simulink model "CAN1_Net_Sim"  (R2026b)
settings: Solver=VariableStepAuto
undefined symbols (not defined in the file or in its folder): P, Ts
libraries: simulink x36
settings Model: Creator=aomar  LastModifiedBy=aomar

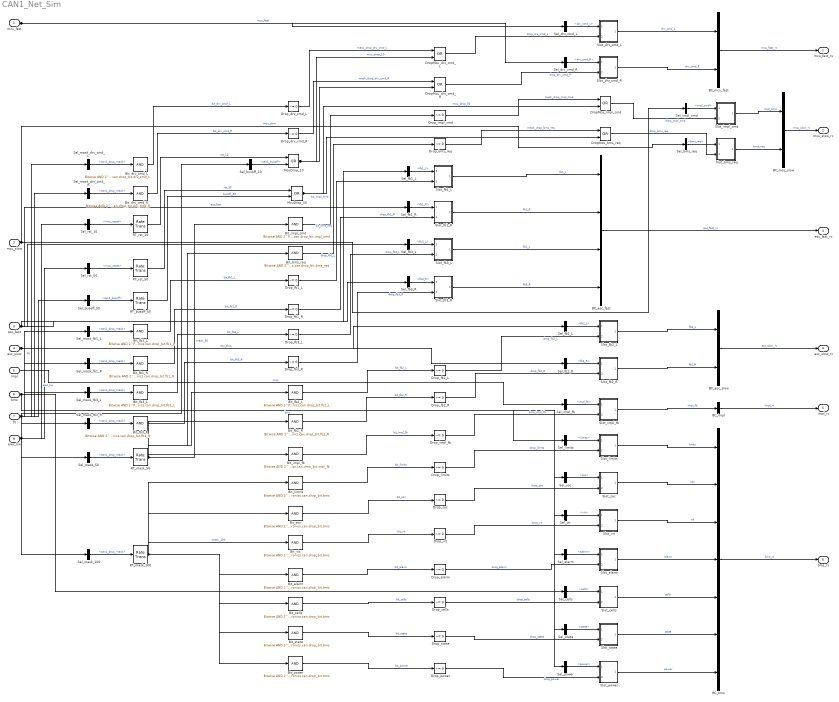
== system CAN1_Net_Sim ==
  mcu_fast : Inport  OutDataTypeStr=Bus: Bus_Can1_McuFast  SampleTime=Ts.ctrl
  mcu_slow : Inport  Port=2  OutDataTypeStr=Bus: Bus_Can1_McuSlow  SampleTime=Ts.comm
  esc_fast : Inport  Port=3  OutDataTypeStr=Bus: Bus_Can1_EscFast  SampleTime=Ts.ctrl
  esc_slow : Inport  Port=4  OutDataTypeStr=Bus: Bus_Can1_EscSlow  SampleTime=Ts.comm
  impl : Inport  Port=5  OutDataTypeStr=Bus: Bus_Can1_Impl  SampleTime=Ts.comm
  bms : Inport  Port=6  OutDataTypeStr=Bus: Bus_Can1_Bms  SampleTime=Ts.hk
  flt : Inport  Port=7  OutDataTypeStr=Bus: Bus_FaultInject  SampleTime=Ts.ctrl
  elec_hw : Inport  Port=8  OutDataTypeStr=Bus: Bus_ElecHwIn  SampleTime=Ts.base
  BC_bms : BusCreator  Inputs=7  OutDataTypeStr=Bus: Bus_Can1_Bms  NonVirtualBus=on
      settings: InheritFromInputs=off
  BC_esc_fast : BusCreator  Inputs=4  OutDataTypeStr=Bus: Bus_Can1_EscFast  NonVirtualBus=on
      settings: InheritFromInputs=off
  BC_esc_slow : BusCreator  Inputs=2  OutDataTypeStr=Bus: Bus_Can1_EscSlow  NonVirtualBus=on
      settings: InheritFromInputs=off
  BC_impl : BusCreator  Inputs=1  OutDataTypeStr=Bus: Bus_Can1_Impl  NonVirtualBus=on
      settings: InheritFromInputs=off
  BC_mcu_fast : BusCreator  Inputs=2  OutDataTypeStr=Bus: Bus_Can1_McuFast  NonVirtualBus=on
      settings: InheritFromInputs=off
  BC_mcu_slow : BusCreator  Inputs=2  OutDataTypeStr=Bus: Bus_Can1_McuSlow  NonVirtualBus=on
      settings: InheritFromInputs=off
  Bit_alarm : simulink/Logic and Bit Operations/Bitwise Operator  logicop=AND  UseBitMask=on  BitMask=2^P.electronics.can.drop_bit.bms  BitMaskRealWorld=Stored Integer
  Bit_bms_req : simulink/Logic and Bit Operations/Bitwise Operator  logicop=AND  UseBitMask=on  BitMask=2^P.electronics.can.drop_bit.bms_req  BitMaskRealWorld=Stored Integer
  Bit_cells : simulink/Logic and Bit Operations/Bitwise Operator  logicop=AND  UseBitMask=on  BitMask=2^P.electronics.can.drop_bit.bms  BitMaskRealWorld=Stored Integer
  Bit_drv_cmd_L : simulink/Logic and Bit Operations/Bitwise Operator  logicop=AND  UseBitMask=on  BitMask=2^P.electronics.can.drop_bit.drv_cmd_L  BitMaskRealWorld=Stored Integer
  Bit_drv_cmd_R : simulink/Logic and Bit Operations/Bitwise Operator  logicop=AND  UseBitMask=on  BitMask=2^P.electronics.can.drop_bit.drv_cmd_R  BitMaskRealWorld=Stored Integer
  Bit_fb1_L : simulink/Logic and Bit Operations/Bitwise Operator  logicop=AND  UseBitMask=on  BitMask=2^P.electronics.can.drop_bit.fb1_L  BitMaskRealWorld=Stored Integer
  Bit_fb1_R : simulink/Logic and Bit Operations/Bitwise Operator  logicop=AND  UseBitMask=on  BitMask=2^P.electronics.can.drop_bit.fb1_R  BitMaskRealWorld=Stored Integer
  Bit_fb2_L : simulink/Logic and Bit Operations/Bitwise Operator  logicop=AND  UseBitMask=on  BitMask=2^P.electronics.can.drop_bit.fb2_L  BitMaskRealWorld=Stored Integer
  Bit_fb2_R : simulink/Logic and Bit Operations/Bitwise Operator  logicop=AND  UseBitMask=on  BitMask=2^P.electronics.can.drop_bit.fb2_R  BitMaskRealWorld=Stored Integer
  Bit_fb3_L : simulink/Logic and Bit Operations/Bitwise Operator  logicop=AND  UseBitMask=on  BitMask=2^P.electronics.can.drop_bit.fb3_L  BitMaskRealWorld=Stored Integer
  Bit_fb3_R : simulink/Logic and Bit Operations/Bitwise Operator  logicop=AND  UseBitMask=on  BitMask=2^P.electronics.can.drop_bit.fb3_R  BitMaskRealWorld=Stored Integer
  Bit_impl_cmd : simulink/Logic and Bit Operations/Bitwise Operator  logicop=AND  UseBitMask=on  BitMask=2^P.electronics.can.drop_bit.impl_cmd  BitMaskRealWorld=Stored Integer
  Bit_impl_fb : simulink/Logic and Bit Operations/Bitwise Operator  logicop=AND  UseBitMask=on  BitMask=2^P.electronics.can.drop_bit.impl_fb  BitMaskRealWorld=Stored Integer
  Bit_limits : simulink/Logic and Bit Operations/Bitwise Operator  logicop=AND  UseBitMask=on  BitMask=2^P.electronics.can.drop_bit.bms  BitMaskRealWorld=Stored Integer
  Bit_power : simulink/Logic and Bit Operations/Bitwise Operator  logicop=AND  UseBitMask=on  BitMask=2^P.electronics.can.drop_bit.bms  BitMaskRealWorld=Stored Integer
  Bit_soc : simulink/Logic and Bit Operations/Bitwise Operator  logicop=AND  UseBitMask=on  BitMask=2^P.electronics.can.drop_bit.bms  BitMaskRealWorld=Stored Integer
  Bit_state : simulink/Logic and Bit Operations/Bitwise Operator  logicop=AND  UseBitMask=on  BitMask=2^P.electronics.can.drop_bit.bms  BitMaskRealWorld=Stored Integer
  Bit_vit : simulink/Logic and Bit Operations/Bitwise Operator  logicop=AND  UseBitMask=on  BitMask=2^P.electronics.can.drop_bit.bms  BitMaskRealWorld=Stored Integer
  DropMcu_bms_req : Logic  Operator=OR  AllPortsSameDT=off  OutDataTypeStr=boolean
  DropMcu_drv_cmd_L : Logic  Operator=OR  AllPortsSameDT=off  OutDataTypeStr=boolean
  DropMcu_drv_cmd_R : Logic  Operator=OR  AllPortsSameDT=off  OutDataTypeStr=boolean
  DropMcu_impl_cmd : Logic  Operator=OR  AllPortsSameDT=off  OutDataTypeStr=boolean
  Drop_alarm : simulink/Logic and Bit Operations/Compare To Zero  relop=~=  OutDataTypeStr=boolean
  Drop_bms_req : simulink/Logic and Bit Operations/Compare To Zero  relop=~=  OutDataTypeStr=boolean
  Drop_cells : simulink/Logic and Bit Operations/Compare To Zero  relop=~=  OutDataTypeStr=boolean
  Drop_drv_cmd_L : simulink/Logic and Bit Operations/Compare To Zero  relop=~=  OutDataTypeStr=boolean
  Drop_drv_cmd_R : simulink/Logic and Bit Operations/Compare To Zero  relop=~=  OutDataTypeStr=boolean
  Drop_fb1_L : simulink/Logic and Bit Operations/Compare To Zero  relop=~=  OutDataTypeStr=boolean
  Drop_fb1_R : simulink/Logic and Bit Operations/Compare To Zero  relop=~=  OutDataTypeStr=boolean
  Drop_fb2_L : simulink/Logic and Bit Operations/Compare To Zero  relop=~=  OutDataTypeStr=boolean
  Drop_fb2_R : simulink/Logic and Bit Operations/Compare To Zero  relop=~=  OutDataTypeStr=boolean
  Drop_fb3_L : simulink/Logic and Bit Operations/Compare To Zero  relop=~=  OutDataTypeStr=boolean
  Drop_fb3_R : simulink/Logic and Bit Operations/Compare To Zero  relop=~=  OutDataTypeStr=boolean
  Drop_impl_cmd : simulink/Logic and Bit Operations/Compare To Zero  relop=~=  OutDataTypeStr=boolean
  Drop_impl_fb : simulink/Logic and Bit Operations/Compare To Zero  relop=~=  OutDataTypeStr=boolean
  Drop_limits : simulink/Logic and Bit Operations/Compare To Zero  relop=~=  OutDataTypeStr=boolean
  Drop_power : simulink/Logic and Bit Operations/Compare To Zero  relop=~=  OutDataTypeStr=boolean
  Drop_soc : simulink/Logic and Bit Operations/Compare To Zero  relop=~=  OutDataTypeStr=boolean
  Drop_state : simulink/Logic and Bit Operations/Compare To Zero  relop=~=  OutDataTypeStr=boolean
  Drop_vit : simulink/Logic and Bit Operations/Compare To Zero  relop=~=  OutDataTypeStr=boolean
  McuDrop_10 : Logic  Operator=OR  AllPortsSameDT=off  OutDataTypeStr=boolean
  McuDrop_50 : Logic  Operator=OR  AllPortsSameDT=off  OutDataTypeStr=boolean
  RT_busoff_50 : RateTransition  InitialCondition=false  OutPortSampleTime=Ts.comm
  RT_mask_100 : RateTransition  OutPortSampleTime=Ts.hk
  RT_mask_50 : RateTransition  OutPortSampleTime=Ts.comm
  RT_rst_10 : RateTransition  InitialCondition=false  OutPortSampleTime=Ts.ctrl
  RT_rst_50 : RateTransition  InitialCondition=false  OutPortSampleTime=Ts.comm
  Sel_alarm : BusSelector  OutputSignals=alarm
  Sel_bms_req : BusSelector  OutputSignals=bms_req
  Sel_busoff_10 : BusSelector  OutputSignals=can1_busoff
  Sel_busoff_50 : BusSelector  OutputSignals=can1_busoff
  Sel_cells : BusSelector  OutputSignals=cells
  Sel_drv_cmd_L : BusSelector  OutputSignals=drv_cmd_L
  Sel_drv_cmd_R : BusSelector  OutputSignals=drv_cmd_R
  Sel_fb1_L : BusSelector  OutputSignals=fb1_L
  Sel_fb1_R : BusSelector  OutputSignals=fb1_R
  Sel_fb2_L : BusSelector  OutputSignals=fb2_L
  Sel_fb2_R : BusSelector  OutputSignals=fb2_R
  Sel_fb3_L : BusSelector  OutputSignals=fb3_L
  Sel_fb3_R : BusSelector  OutputSignals=fb3_R
  Sel_impl_cmd : BusSelector  OutputSignals=impl_cmd
  Sel_impl_fb : BusSelector  OutputSignals=impl_fb
  Sel_limits : BusSelector  OutputSignals=limits
  Sel_mask_100 : BusSelector  OutputSignals=can1_drop_mask
  Sel_mask_50 : BusSelector  OutputSignals=can1_drop_mask
  Sel_mask_drv_cmd_L : BusSelector  OutputSignals=can1_drop_mask
  Sel_mask_drv_cmd_R : BusSelector  OutputSignals=can1_drop_mask
  Sel_mask_fb1_L : BusSelector  OutputSignals=can1_drop_mask
  Sel_mask_fb1_R : BusSelector  OutputSignals=can1_drop_mask
  Sel_mask_fb3_L : BusSelector  OutputSignals=can1_drop_mask
  Sel_mask_fb3_R : BusSelector  OutputSignals=can1_drop_mask
  Sel_power : BusSelector  OutputSignals=power
  Sel_rst_10 : BusSelector  OutputSignals=mcu_reset
  Sel_rst_50 : BusSelector  OutputSignals=mcu_reset
  Sel_soc : BusSelector  OutputSignals=soc
  Sel_state : BusSelector  OutputSignals=state
  Sel_vit : BusSelector  OutputSignals=vit
  Slot_alarm : Subsystem
  Slot_bms_req : Subsystem
  Slot_cells : Subsystem
  Slot_drv_cmd_L : Subsystem
  Slot_drv_cmd_R : Subsystem
  Slot_fb1_L : Subsystem
  Slot_fb1_R : Subsystem
  Slot_fb2_L : Subsystem
  Slot_fb2_R : Subsystem
  Slot_fb3_L : Subsystem
  Slot_fb3_R : Subsystem
  Slot_impl_cmd : Subsystem
  Slot_impl_fb : Subsystem
  Slot_limits : Subsystem
  Slot_power : Subsystem
  Slot_soc : Subsystem
  Slot_state : Subsystem
  Slot_vit : Subsystem
  mcu_fast_rx : Outport  OutDataTypeStr=Bus: Bus_Can1_McuFast
  mcu_slow_rx : Outport  Port=2  OutDataTypeStr=Bus: Bus_Can1_McuSlow
  esc_fast_rx : Outport  Port=3  OutDataTypeStr=Bus: Bus_Can1_EscFast
  esc_slow_rx : Outport  Port=4  OutDataTypeStr=Bus: Bus_Can1_EscSlow
  impl_rx : Outport  Port=5  OutDataTypeStr=Bus: Bus_Can1_Impl
  bms_rx : Outport  Port=6  OutDataTypeStr=Bus: Bus_Can1_Bms
  wires:
  mcu_fast/1 -> Sel_drv_cmd_R/1, Sel_drv_cmd_L/1  "mcu_fast"
  mcu_slow/1 -> Sel_impl_cmd/1, Sel_bms_req/1  "mcu_slow"
  esc_fast/1 -> Sel_fb1_L/1, Sel_fb1_R/1, Sel_fb3_L/1, Sel_fb3_R/1  "esc_fast"
  esc_slow/1 -> Sel_fb2_L/1, Sel_fb2_R/1  "esc_slow"
  impl/1 -> Sel_impl_fb/1  "impl"
  elec_hw/1 -> Sel_rst_10/1, Sel_rst_50/1  "elec_hw"
  Sel_mask_drv_cmd_L/1 -> Bit_drv_cmd_L/1  "<can1_drop_mask>"
  Sel_mask_drv_cmd_R/1 -> Bit_drv_cmd_R/1  "<can1_drop_mask>"
  Sel_rst_10/1 -> RT_rst_10/1  "<mcu_reset>"
  Sel_rst_50/1 -> RT_rst_50/1  "<mcu_reset>"
  Sel_busoff_50/1 -> RT_busoff_50/1  "<can1_busoff>"
  Sel_mask_fb1_L/1 -> Bit_fb1_L/1  "<can1_drop_mask>"
  Sel_mask_fb1_R/1 -> Bit_fb1_R/1  "<can1_drop_mask>"
  Sel_mask_fb3_L/1 -> Bit_fb3_L/1  "<can1_drop_mask>"
  Sel_mask_fb3_R/1 -> Bit_fb3_R/1  "<can1_drop_mask>"
  Sel_mask_50/1 -> RT_mask_50/1  "<can1_drop_mask>"
  Sel_mask_100/1 -> RT_mask_100/1  "<can1_drop_mask>"
  Bit_drv_cmd_L/1 -> Drop_drv_cmd_L/1  "bit_drv_cmd_L"
  Bit_drv_cmd_R/1 -> Drop_drv_cmd_R/1  "bit_drv_cmd_R"
  RT_rst_10/1 -> McuDrop_10/1  "rst_10"
  RT_rst_50/1 -> McuDrop_50/1  "rst_50"
  RT_busoff_50/1 -> McuDrop_50/2  "busoff_50"
  Bit_fb1_L/1 -> Drop_fb1_L/1  "bit_fb1_L"
  Bit_fb1_R/1 -> Drop_fb1_R/1  "bit_fb1_R"
  Bit_fb3_L/1 -> Drop_fb3_L/1  "bit_fb3_L"
  Bit_fb3_R/1 -> Drop_fb3_R/1  "bit_fb3_R"
  RT_mask_50/1 -> Bit_impl_cmd/1, Bit_bms_req/1, Bit_fb2_L/1, Bit_fb2_R/1, Bit_impl_fb/1  "mask_50"
  RT_mask_100/1 -> Bit_power/1, Bit_state/1, Bit_limits/1, Bit_cells/1, Bit_soc/1, Bit_alarm/1, Bit_vit/1  "mask_100"
  Sel_busoff_10/1 -> McuDrop_10/2  "<can1_busoff>"
  Drop_drv_cmd_L/1 -> DropMcu_drv_cmd_L/1  "mask_drop_drv_cmd_L"
  Drop_drv_cmd_R/1 -> DropMcu_drv_cmd_R/1  "mask_drop_drv_cmd_R"
  McuDrop_10/1 -> DropMcu_drv_cmd_L/2, DropMcu_drv_cmd_R/2  "mcu_drop_10"
  Drop_fb1_L/1 -> Slot_fb1_L/2(drop)  "drop_fb1_L"
  Drop_fb1_R/1 -> Slot_fb1_R/2(drop)  "drop_fb1_R"
  Drop_fb3_L/1 -> Slot_fb3_L/2(drop)  "drop_fb3_L"
  Drop_fb3_R/1 -> Slot_fb3_R/2(drop)  "drop_fb3_R"
  McuDrop_50/1 -> DropMcu_impl_cmd/2, DropMcu_bms_req/2  "mcu_drop_50"
  Bit_impl_cmd/1 -> Drop_impl_cmd/1  "bit_impl_cmd"
  Bit_bms_req/1 -> Drop_bms_req/1  "bit_bms_req"
  Bit_fb2_L/1 -> Drop_fb2_L/1  "bit_fb2_L"
  Bit_fb2_R/1 -> Drop_fb2_R/1  "bit_fb2_R"
  Bit_impl_fb/1 -> Drop_impl_fb/1  "bit_impl_fb"
  Bit_limits/1 -> Drop_limits/1  "bit_limits"
  Bit_soc/1 -> Drop_soc/1  "bit_soc"
  Bit_vit/1 -> Drop_vit/1  "bit_vit"
  Bit_alarm/1 -> Drop_alarm/1  "bit_alarm"
  Bit_cells/1 -> Drop_cells/1  "bit_cells"
  Bit_state/1 -> Drop_state/1  "bit_state"
  Bit_power/1 -> Drop_power/1  "bit_power"
  Sel_fb1_L/1 -> Slot_fb1_L/1(frame)  "<fb1_L>"
  Sel_fb1_R/1 -> Slot_fb1_R/1(frame)  "<fb1_R>"
  Sel_fb3_L/1 -> Slot_fb3_L/1(frame)  "<fb3_L>"
  Sel_fb3_R/1 -> Slot_fb3_R/1(frame)  "<fb3_R>"
  DropMcu_drv_cmd_L/1 -> Slot_drv_cmd_L/2(drop)  "drop_drv_cmd_L"
  DropMcu_drv_cmd_R/1 -> Slot_drv_cmd_R/2(drop)  "drop_drv_cmd_R"
  Drop_impl_cmd/1 -> DropMcu_impl_cmd/1  "mask_drop_impl_cmd"
  Drop_bms_req/1 -> DropMcu_bms_req/1  "mask_drop_bms_req"
  Drop_fb2_L/1 -> Slot_fb2_L/2(drop)  "drop_fb2_L"
  Drop_fb2_R/1 -> Slot_fb2_R/2(drop)  "drop_fb2_R"
  Drop_impl_fb/1 -> Slot_impl_fb/2(drop)  "drop_impl_fb"
  Drop_limits/1 -> Slot_limits/2(drop)  "drop_limits"
  Drop_soc/1 -> Slot_soc/2(drop)  "drop_soc"
  Drop_vit/1 -> Slot_vit/2(drop)  "drop_vit"
  Drop_alarm/1 -> Slot_alarm/2(drop)  "drop_alarm"
  Drop_cells/1 -> Slot_cells/2(drop)  "drop_cells"
  Drop_state/1 -> Slot_state/2(drop)  "drop_state"
  Drop_power/1 -> Slot_power/2(drop)  "drop_power"
  Slot_fb1_L/1(frame_rx) -> BC_esc_fast/1  "fb1_L"
  Slot_fb1_R/1(frame_rx) -> BC_esc_fast/2  "fb1_R"
  Slot_fb3_L/1(frame_rx) -> BC_esc_fast/3  "fb3_L"
  Slot_fb3_R/1(frame_rx) -> BC_esc_fast/4  "fb3_R"
  Sel_drv_cmd_L/1 -> Slot_drv_cmd_L/1(frame)  "<drv_cmd_L>"
  Sel_drv_cmd_R/1 -> Slot_drv_cmd_R/1(frame)  "<drv_cmd_R>"
  Sel_fb2_L/1 -> Slot_fb2_L/1(frame)  "<fb2_L>"
  Sel_fb2_R/1 -> Slot_fb2_R/1(frame)  "<fb2_R>"
  Sel_impl_fb/1 -> Slot_impl_fb/1(frame)  "<impl_fb>"
  Sel_limits/1 -> Slot_limits/1(frame)  "<limits>"
  Sel_soc/1 -> Slot_soc/1(frame)  "<soc>"
  Sel_vit/1 -> Slot_vit/1(frame)  "<vit>"
  Sel_alarm/1 -> Slot_alarm/1(frame)  "<alarm>"
  Sel_cells/1 -> Slot_cells/1(frame)  "<cells>"
  Sel_state/1 -> Slot_state/1(frame)  "<state>"
  Sel_power/1 -> Slot_power/1(frame)  "<power>"
  BC_esc_fast/1 -> esc_fast_rx/1  "esc_fast_rx"
  DropMcu_impl_cmd/1 -> Slot_impl_cmd/2(drop)  "drop_impl_cmd"
  DropMcu_bms_req/1 -> Slot_bms_req/2(drop)  "drop_bms_req"
  Slot_drv_cmd_L/1(frame_rx) -> BC_mcu_fast/1  "drv_cmd_L"
  Slot_drv_cmd_R/1(frame_rx) -> BC_mcu_fast/2  "drv_cmd_R"
  Slot_fb2_L/1(frame_rx) -> BC_esc_slow/1  "fb2_L"
  Slot_fb2_R/1(frame_rx) -> BC_esc_slow/2  "fb2_R"
  Slot_impl_fb/1(frame_rx) -> BC_impl/1  "impl_fb"
  Slot_limits/1(frame_rx) -> BC_bms/1  "limits"
  Slot_soc/1(frame_rx) -> BC_bms/2  "soc"
  Slot_vit/1(frame_rx) -> BC_bms/3  "vit"
  Slot_alarm/1(frame_rx) -> BC_bms/4  "alarm"
  Slot_cells/1(frame_rx) -> BC_bms/5  "cells"
  Slot_state/1(frame_rx) -> BC_bms/6  "state"
  Slot_power/1(frame_rx) -> BC_bms/7  "power"
  Sel_impl_cmd/1 -> Slot_impl_cmd/1(frame)  "<impl_cmd>"
  Sel_bms_req/1 -> Slot_bms_req/1(frame)  "<bms_req>"
  BC_mcu_fast/1 -> mcu_fast_rx/1  "mcu_fast_rx"
  BC_esc_slow/1 -> esc_slow_rx/1  "esc_slow_rx"
  BC_impl/1 -> impl_rx/1  "impl_rx"
  BC_bms/1 -> bms_rx/1  "bms_rx"
  Slot_impl_cmd/1(frame_rx) -> BC_mcu_slow/1  "impl_cmd"
  Slot_bms_req/1(frame_rx) -> BC_mcu_slow/2  "bms_req"
  BC_mcu_slow/1 -> mcu_slow_rx/1  "mcu_slow_rx"
  bms/1 -> Sel_cells/1, Sel_power/1, Sel_state/1, Sel_alarm/1, Sel_vit/1, Sel_soc/1, Sel_limits/1  "bms"
  flt/1 -> Sel_mask_drv_cmd_L/1, Sel_busoff_10/1, Sel_mask_drv_cmd_R/1, Sel_mask_100/1, Sel_busoff_50/1, Sel_mask_fb1_L/1, Sel_mask_fb1_R/1, Sel_mask_50/1, Sel_mask_fb3_L/1, Sel_mask_fb3_R/1  "flt"

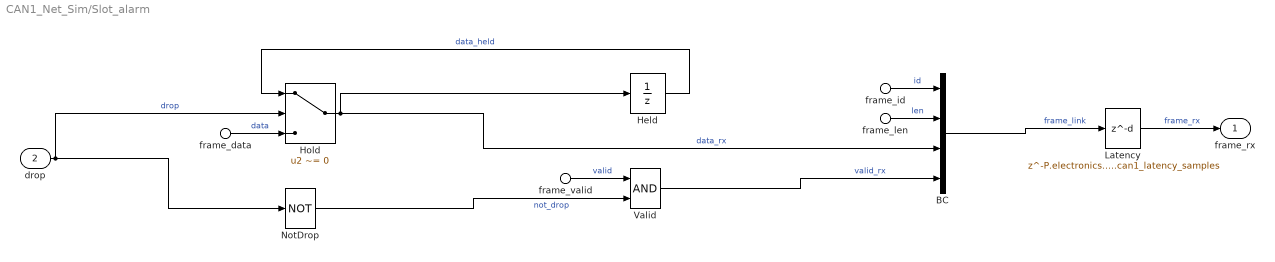
== system CAN1_Net_Sim/Slot_alarm ==
  frame_id : Inport  PortName=frame  Element=id
  frame_len : Inport  PortName=frame  Element=len
  frame_data : Inport  PortName=frame  Element=data
  frame_valid : Inport  PortName=frame  Element=valid
  drop : Inport  Port=2
  BC : BusCreator  Inputs=4  OutDataTypeStr=Bus: Bus_CanFrame8  NonVirtualBus=on
      settings: InheritFromInputs=off
  Held : UnitDelay  SampleTime=Ts.hk
  Hold : Switch  Criteria=u2 ~= 0  SaturateOnIntegerOverflow=off  InputSameDT=off
  Latency : Delay  DelayLength=P.electronics.can.can1_latency_samples  InitialCondition=P.ic.Bus_CanFrame8  SampleTime=Ts.hk
  NotDrop : Logic  Operator=NOT  Inputs=1  AllPortsSameDT=off  OutDataTypeStr=boolean
  Valid : Logic  AllPortsSameDT=off  OutDataTypeStr=boolean
  frame_rx : Outport
  wires:
  drop/1 -> NotDrop/1, Hold/2  "drop"
  frame_data/1 -> Hold/3  "data"
  NotDrop/1 -> Valid/2  "not_drop"
  Hold/1 -> BC/3, Held/1  "data_rx"
  frame_valid/1 -> Valid/1  "valid"
  Valid/1 -> BC/4  "valid_rx"
  Held/1 -> Hold/1  "data_held"
  frame_id/1 -> BC/1  "id"
  frame_len/1 -> BC/2  "len"
  BC/1 -> Latency/1  "frame_link"
  Latency/1 -> frame_rx/1  "frame_rx"

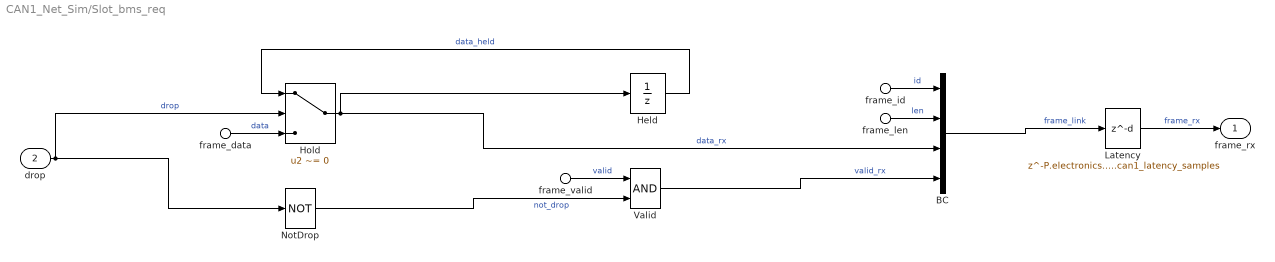
== system CAN1_Net_Sim/Slot_bms_req ==
  frame_id : Inport  PortName=frame  Element=id
  frame_len : Inport  PortName=frame  Element=len
  frame_data : Inport  PortName=frame  Element=data
  frame_valid : Inport  PortName=frame  Element=valid
  drop : Inport  Port=2
  BC : BusCreator  Inputs=4  OutDataTypeStr=Bus: Bus_CanFrame8  NonVirtualBus=on
      settings: InheritFromInputs=off
  Held : UnitDelay  SampleTime=Ts.comm
  Hold : Switch  Criteria=u2 ~= 0  SaturateOnIntegerOverflow=off  InputSameDT=off
  Latency : Delay  DelayLength=P.electronics.can.can1_latency_samples  InitialCondition=P.ic.Bus_CanFrame8  SampleTime=Ts.comm
  NotDrop : Logic  Operator=NOT  Inputs=1  AllPortsSameDT=off  OutDataTypeStr=boolean
  Valid : Logic  AllPortsSameDT=off  OutDataTypeStr=boolean
  frame_rx : Outport
  wires:
  drop/1 -> NotDrop/1, Hold/2  "drop"
  frame_data/1 -> Hold/3  "data"
  NotDrop/1 -> Valid/2  "not_drop"
  Hold/1 -> BC/3, Held/1  "data_rx"
  frame_valid/1 -> Valid/1  "valid"
  Valid/1 -> BC/4  "valid_rx"
  Held/1 -> Hold/1  "data_held"
  frame_id/1 -> BC/1  "id"
  frame_len/1 -> BC/2  "len"
  BC/1 -> Latency/1  "frame_link"
  Latency/1 -> frame_rx/1  "frame_rx"

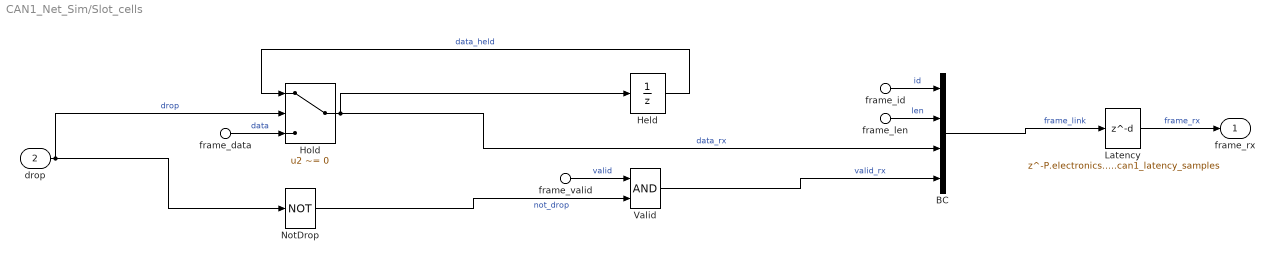
== system CAN1_Net_Sim/Slot_cells ==
  frame_id : Inport  PortName=frame  Element=id
  frame_len : Inport  PortName=frame  Element=len
  frame_data : Inport  PortName=frame  Element=data
  frame_valid : Inport  PortName=frame  Element=valid
  drop : Inport  Port=2
  BC : BusCreator  Inputs=4  OutDataTypeStr=Bus: Bus_CanFrame8  NonVirtualBus=on
      settings: InheritFromInputs=off
  Held : UnitDelay  SampleTime=Ts.hk
  Hold : Switch  Criteria=u2 ~= 0  SaturateOnIntegerOverflow=off  InputSameDT=off
  Latency : Delay  DelayLength=P.electronics.can.can1_latency_samples  InitialCondition=P.ic.Bus_CanFrame8  SampleTime=Ts.hk
  NotDrop : Logic  Operator=NOT  Inputs=1  AllPortsSameDT=off  OutDataTypeStr=boolean
  Valid : Logic  AllPortsSameDT=off  OutDataTypeStr=boolean
  frame_rx : Outport
  wires:
  drop/1 -> NotDrop/1, Hold/2  "drop"
  frame_data/1 -> Hold/3  "data"
  NotDrop/1 -> Valid/2  "not_drop"
  Hold/1 -> BC/3, Held/1  "data_rx"
  frame_valid/1 -> Valid/1  "valid"
  Valid/1 -> BC/4  "valid_rx"
  Held/1 -> Hold/1  "data_held"
  frame_id/1 -> BC/1  "id"
  frame_len/1 -> BC/2  "len"
  BC/1 -> Latency/1  "frame_link"
  Latency/1 -> frame_rx/1  "frame_rx"

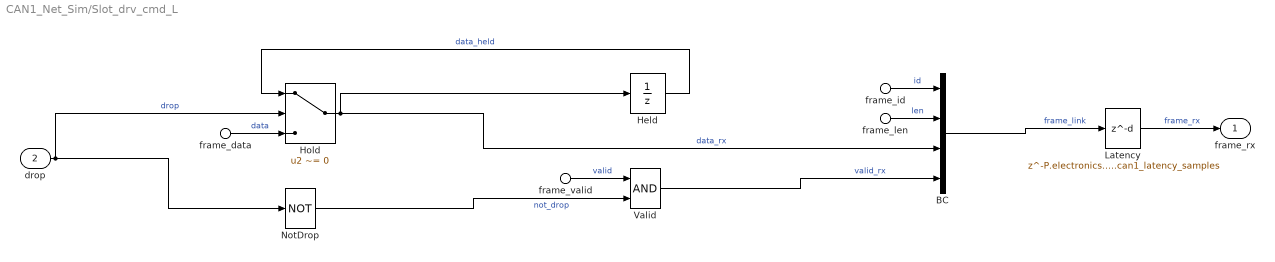
== system CAN1_Net_Sim/Slot_drv_cmd_L ==
  frame_id : Inport  PortName=frame  Element=id
  frame_len : Inport  PortName=frame  Element=len
  frame_data : Inport  PortName=frame  Element=data
  frame_valid : Inport  PortName=frame  Element=valid
  drop : Inport  Port=2
  BC : BusCreator  Inputs=4  OutDataTypeStr=Bus: Bus_CanFrame8  NonVirtualBus=on
      settings: InheritFromInputs=off
  Held : UnitDelay  SampleTime=Ts.ctrl
  Hold : Switch  Criteria=u2 ~= 0  SaturateOnIntegerOverflow=off  InputSameDT=off
  Latency : Delay  DelayLength=P.electronics.can.can1_latency_samples  InitialCondition=P.ic.Bus_CanFrame8  SampleTime=Ts.ctrl
  NotDrop : Logic  Operator=NOT  Inputs=1  AllPortsSameDT=off  OutDataTypeStr=boolean
  Valid : Logic  AllPortsSameDT=off  OutDataTypeStr=boolean
  frame_rx : Outport
  wires:
  drop/1 -> NotDrop/1, Hold/2  "drop"
  frame_data/1 -> Hold/3  "data"
  NotDrop/1 -> Valid/2  "not_drop"
  Hold/1 -> BC/3, Held/1  "data_rx"
  frame_valid/1 -> Valid/1  "valid"
  Valid/1 -> BC/4  "valid_rx"
  Held/1 -> Hold/1  "data_held"
  frame_id/1 -> BC/1  "id"
  frame_len/1 -> BC/2  "len"
  BC/1 -> Latency/1  "frame_link"
  Latency/1 -> frame_rx/1  "frame_rx"

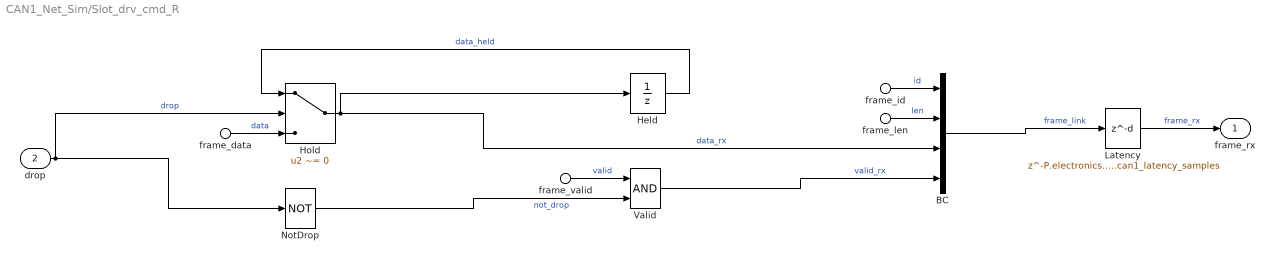
== system CAN1_Net_Sim/Slot_drv_cmd_R ==
  frame_id : Inport  PortName=frame  Element=id
  frame_len : Inport  PortName=frame  Element=len
  frame_data : Inport  PortName=frame  Element=data
  frame_valid : Inport  PortName=frame  Element=valid
  drop : Inport  Port=2
  BC : BusCreator  Inputs=4  OutDataTypeStr=Bus: Bus_CanFrame8  NonVirtualBus=on
      settings: InheritFromInputs=off
  Held : UnitDelay  SampleTime=Ts.ctrl
  Hold : Switch  Criteria=u2 ~= 0  SaturateOnIntegerOverflow=off  InputSameDT=off
  Latency : Delay  DelayLength=P.electronics.can.can1_latency_samples  InitialCondition=P.ic.Bus_CanFrame8  SampleTime=Ts.ctrl
  NotDrop : Logic  Operator=NOT  Inputs=1  AllPortsSameDT=off  OutDataTypeStr=boolean
  Valid : Logic  AllPortsSameDT=off  OutDataTypeStr=boolean
  frame_rx : Outport
  wires:
  drop/1 -> NotDrop/1, Hold/2  "drop"
  frame_data/1 -> Hold/3  "data"
  NotDrop/1 -> Valid/2  "not_drop"
  Hold/1 -> BC/3, Held/1  "data_rx"
  frame_valid/1 -> Valid/1  "valid"
  Valid/1 -> BC/4  "valid_rx"
  Held/1 -> Hold/1  "data_held"
  frame_id/1 -> BC/1  "id"
  frame_len/1 -> BC/2  "len"
  BC/1 -> Latency/1  "frame_link"
  Latency/1 -> frame_rx/1  "frame_rx"

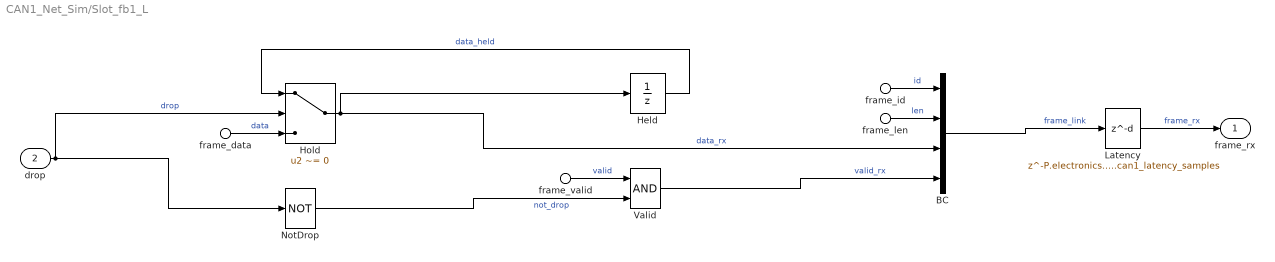
== system CAN1_Net_Sim/Slot_fb1_L ==
  frame_id : Inport  PortName=frame  Element=id
  frame_len : Inport  PortName=frame  Element=len
  frame_data : Inport  PortName=frame  Element=data
  frame_valid : Inport  PortName=frame  Element=valid
  drop : Inport  Port=2
  BC : BusCreator  Inputs=4  OutDataTypeStr=Bus: Bus_CanFrame8  NonVirtualBus=on
      settings: InheritFromInputs=off
  Held : UnitDelay  SampleTime=Ts.ctrl
  Hold : Switch  Criteria=u2 ~= 0  SaturateOnIntegerOverflow=off  InputSameDT=off
  Latency : Delay  DelayLength=P.electronics.can.can1_latency_samples  InitialCondition=P.ic.Bus_CanFrame8  SampleTime=Ts.ctrl
  NotDrop : Logic  Operator=NOT  Inputs=1  AllPortsSameDT=off  OutDataTypeStr=boolean
  Valid : Logic  AllPortsSameDT=off  OutDataTypeStr=boolean
  frame_rx : Outport
  wires:
  drop/1 -> NotDrop/1, Hold/2  "drop"
  frame_data/1 -> Hold/3  "data"
  NotDrop/1 -> Valid/2  "not_drop"
  Hold/1 -> BC/3, Held/1  "data_rx"
  frame_valid/1 -> Valid/1  "valid"
  Valid/1 -> BC/4  "valid_rx"
  Held/1 -> Hold/1  "data_held"
  frame_id/1 -> BC/1  "id"
  frame_len/1 -> BC/2  "len"
  BC/1 -> Latency/1  "frame_link"
  Latency/1 -> frame_rx/1  "frame_rx"

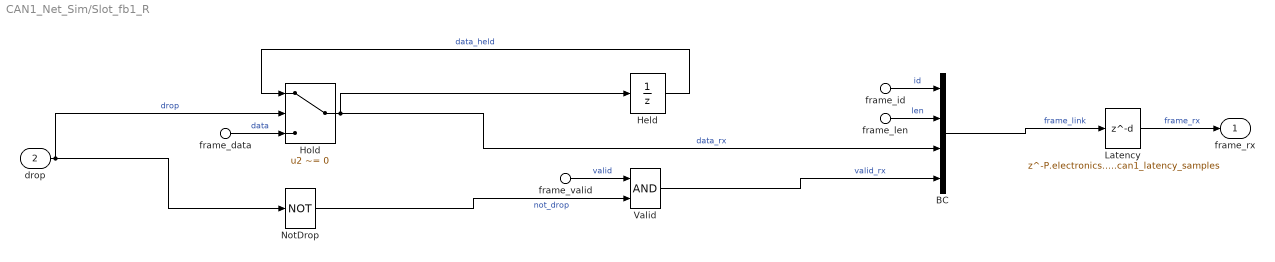
== system CAN1_Net_Sim/Slot_fb1_R ==
  frame_id : Inport  PortName=frame  Element=id
  frame_len : Inport  PortName=frame  Element=len
  frame_data : Inport  PortName=frame  Element=data
  frame_valid : Inport  PortName=frame  Element=valid
  drop : Inport  Port=2
  BC : BusCreator  Inputs=4  OutDataTypeStr=Bus: Bus_CanFrame8  NonVirtualBus=on
      settings: InheritFromInputs=off
  Held : UnitDelay  SampleTime=Ts.ctrl
  Hold : Switch  Criteria=u2 ~= 0  SaturateOnIntegerOverflow=off  InputSameDT=off
  Latency : Delay  DelayLength=P.electronics.can.can1_latency_samples  InitialCondition=P.ic.Bus_CanFrame8  SampleTime=Ts.ctrl
  NotDrop : Logic  Operator=NOT  Inputs=1  AllPortsSameDT=off  OutDataTypeStr=boolean
  Valid : Logic  AllPortsSameDT=off  OutDataTypeStr=boolean
  frame_rx : Outport
  wires:
  drop/1 -> NotDrop/1, Hold/2  "drop"
  frame_data/1 -> Hold/3  "data"
  NotDrop/1 -> Valid/2  "not_drop"
  Hold/1 -> BC/3, Held/1  "data_rx"
  frame_valid/1 -> Valid/1  "valid"
  Valid/1 -> BC/4  "valid_rx"
  Held/1 -> Hold/1  "data_held"
  frame_id/1 -> BC/1  "id"
  frame_len/1 -> BC/2  "len"
  BC/1 -> Latency/1  "frame_link"
  Latency/1 -> frame_rx/1  "frame_rx"

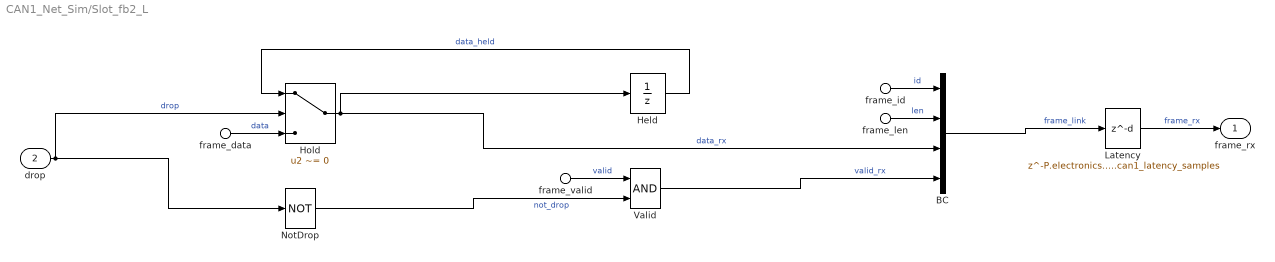
== system CAN1_Net_Sim/Slot_fb2_L ==
  frame_id : Inport  PortName=frame  Element=id
  frame_len : Inport  PortName=frame  Element=len
  frame_data : Inport  PortName=frame  Element=data
  frame_valid : Inport  PortName=frame  Element=valid
  drop : Inport  Port=2
  BC : BusCreator  Inputs=4  OutDataTypeStr=Bus: Bus_CanFrame8  NonVirtualBus=on
      settings: InheritFromInputs=off
  Held : UnitDelay  SampleTime=Ts.comm
  Hold : Switch  Criteria=u2 ~= 0  SaturateOnIntegerOverflow=off  InputSameDT=off
  Latency : Delay  DelayLength=P.electronics.can.can1_latency_samples  InitialCondition=P.ic.Bus_CanFrame8  SampleTime=Ts.comm
  NotDrop : Logic  Operator=NOT  Inputs=1  AllPortsSameDT=off  OutDataTypeStr=boolean
  Valid : Logic  AllPortsSameDT=off  OutDataTypeStr=boolean
  frame_rx : Outport
  wires:
  drop/1 -> NotDrop/1, Hold/2  "drop"
  frame_data/1 -> Hold/3  "data"
  NotDrop/1 -> Valid/2  "not_drop"
  Hold/1 -> BC/3, Held/1  "data_rx"
  frame_valid/1 -> Valid/1  "valid"
  Valid/1 -> BC/4  "valid_rx"
  Held/1 -> Hold/1  "data_held"
  frame_id/1 -> BC/1  "id"
  frame_len/1 -> BC/2  "len"
  BC/1 -> Latency/1  "frame_link"
  Latency/1 -> frame_rx/1  "frame_rx"

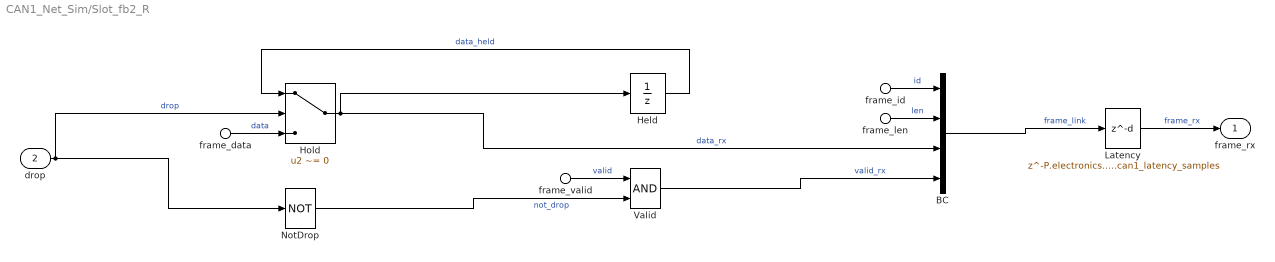
== system CAN1_Net_Sim/Slot_fb2_R ==
  frame_id : Inport  PortName=frame  Element=id
  frame_len : Inport  PortName=frame  Element=len
  frame_data : Inport  PortName=frame  Element=data
  frame_valid : Inport  PortName=frame  Element=valid
  drop : Inport  Port=2
  BC : BusCreator  Inputs=4  OutDataTypeStr=Bus: Bus_CanFrame8  NonVirtualBus=on
      settings: InheritFromInputs=off
  Held : UnitDelay  SampleTime=Ts.comm
  Hold : Switch  Criteria=u2 ~= 0  SaturateOnIntegerOverflow=off  InputSameDT=off
  Latency : Delay  DelayLength=P.electronics.can.can1_latency_samples  InitialCondition=P.ic.Bus_CanFrame8  SampleTime=Ts.comm
  NotDrop : Logic  Operator=NOT  Inputs=1  AllPortsSameDT=off  OutDataTypeStr=boolean
  Valid : Logic  AllPortsSameDT=off  OutDataTypeStr=boolean
  frame_rx : Outport
  wires:
  drop/1 -> NotDrop/1, Hold/2  "drop"
  frame_data/1 -> Hold/3  "data"
  NotDrop/1 -> Valid/2  "not_drop"
  Hold/1 -> BC/3, Held/1  "data_rx"
  frame_valid/1 -> Valid/1  "valid"
  Valid/1 -> BC/4  "valid_rx"
  Held/1 -> Hold/1  "data_held"
  frame_id/1 -> BC/1  "id"
  frame_len/1 -> BC/2  "len"
  BC/1 -> Latency/1  "frame_link"
  Latency/1 -> frame_rx/1  "frame_rx"

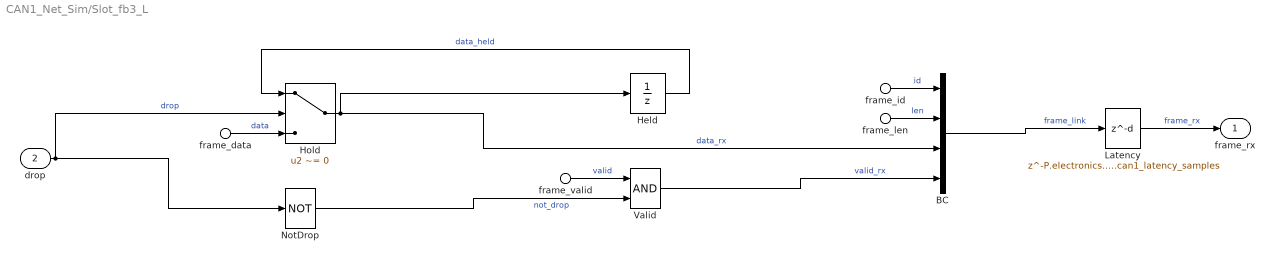
== system CAN1_Net_Sim/Slot_fb3_L ==
  frame_id : Inport  PortName=frame  Element=id
  frame_len : Inport  PortName=frame  Element=len
  frame_data : Inport  PortName=frame  Element=data
  frame_valid : Inport  PortName=frame  Element=valid
  drop : Inport  Port=2
  BC : BusCreator  Inputs=4  OutDataTypeStr=Bus: Bus_CanFrame8  NonVirtualBus=on
      settings: InheritFromInputs=off
  Held : UnitDelay  SampleTime=Ts.ctrl
  Hold : Switch  Criteria=u2 ~= 0  SaturateOnIntegerOverflow=off  InputSameDT=off
  Latency : Delay  DelayLength=P.electronics.can.can1_latency_samples  InitialCondition=P.ic.Bus_CanFrame8  SampleTime=Ts.ctrl
  NotDrop : Logic  Operator=NOT  Inputs=1  AllPortsSameDT=off  OutDataTypeStr=boolean
  Valid : Logic  AllPortsSameDT=off  OutDataTypeStr=boolean
  frame_rx : Outport
  wires:
  drop/1 -> NotDrop/1, Hold/2  "drop"
  frame_data/1 -> Hold/3  "data"
  NotDrop/1 -> Valid/2  "not_drop"
  Hold/1 -> BC/3, Held/1  "data_rx"
  frame_valid/1 -> Valid/1  "valid"
  Valid/1 -> BC/4  "valid_rx"
  Held/1 -> Hold/1  "data_held"
  frame_id/1 -> BC/1  "id"
  frame_len/1 -> BC/2  "len"
  BC/1 -> Latency/1  "frame_link"
  Latency/1 -> frame_rx/1  "frame_rx"

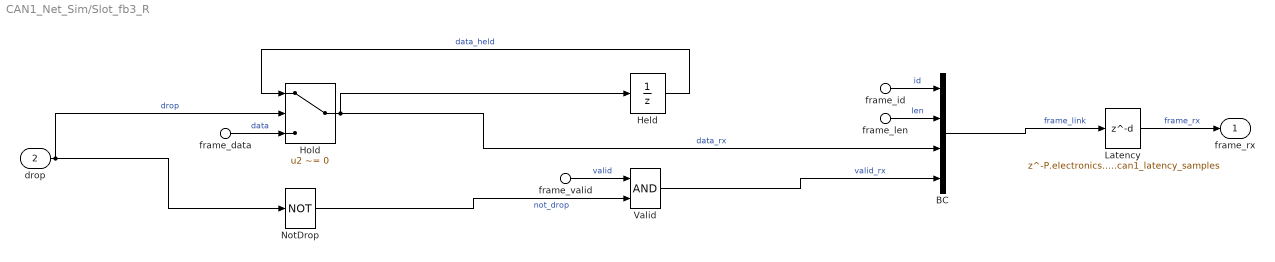
== system CAN1_Net_Sim/Slot_fb3_R ==
  frame_id : Inport  PortName=frame  Element=id
  frame_len : Inport  PortName=frame  Element=len
  frame_data : Inport  PortName=frame  Element=data
  frame_valid : Inport  PortName=frame  Element=valid
  drop : Inport  Port=2
  BC : BusCreator  Inputs=4  OutDataTypeStr=Bus: Bus_CanFrame8  NonVirtualBus=on
      settings: InheritFromInputs=off
  Held : UnitDelay  SampleTime=Ts.ctrl
  Hold : Switch  Criteria=u2 ~= 0  SaturateOnIntegerOverflow=off  InputSameDT=off
  Latency : Delay  DelayLength=P.electronics.can.can1_latency_samples  InitialCondition=P.ic.Bus_CanFrame8  SampleTime=Ts.ctrl
  NotDrop : Logic  Operator=NOT  Inputs=1  AllPortsSameDT=off  OutDataTypeStr=boolean
  Valid : Logic  AllPortsSameDT=off  OutDataTypeStr=boolean
  frame_rx : Outport
  wires:
  drop/1 -> NotDrop/1, Hold/2  "drop"
  frame_data/1 -> Hold/3  "data"
  NotDrop/1 -> Valid/2  "not_drop"
  Hold/1 -> BC/3, Held/1  "data_rx"
  frame_valid/1 -> Valid/1  "valid"
  Valid/1 -> BC/4  "valid_rx"
  Held/1 -> Hold/1  "data_held"
  frame_id/1 -> BC/1  "id"
  frame_len/1 -> BC/2  "len"
  BC/1 -> Latency/1  "frame_link"
  Latency/1 -> frame_rx/1  "frame_rx"

== system CAN1_Net_Sim/Slot_impl_cmd ==
  frame_id : Inport  PortName=frame  Element=id
  frame_len : Inport  PortName=frame  Element=len
  frame_data : Inport  PortName=frame  Element=data
  frame_valid : Inport  PortName=frame  Element=valid
  drop : Inport  Port=2
  BC : BusCreator  Inputs=4  OutDataTypeStr=Bus: Bus_CanFrame8  NonVirtualBus=on
      settings: InheritFromInputs=off
  Held : UnitDelay  SampleTime=Ts.comm
  Hold : Switch  Criteria=u2 ~= 0  SaturateOnIntegerOverflow=off  InputSameDT=off
  Latency : Delay  DelayLength=P.electronics.can.can1_latency_samples  InitialCondition=P.ic.Bus_CanFrame8  SampleTime=Ts.comm
  NotDrop : Logic  Operator=NOT  Inputs=1  AllPortsSameDT=off  OutDataTypeStr=boolean
  Valid : Logic  AllPortsSameDT=off  OutDataTypeStr=boolean
  frame_rx : Outport
  wires:
  drop/1 -> NotDrop/1, Hold/2  "drop"
  frame_data/1 -> Hold/3  "data"
  NotDrop/1 -> Valid/2  "not_drop"
  Hold/1 -> BC/3, Held/1  "data_rx"
  frame_valid/1 -> Valid/1  "valid"
  Valid/1 -> BC/4  "valid_rx"
  Held/1 -> Hold/1  "data_held"
  frame_id/1 -> BC/1  "id"
  frame_len/1 -> BC/2  "len"
  BC/1 -> Latency/1  "frame_link"
  Latency/1 -> frame_rx/1  "frame_rx"

== system CAN1_Net_Sim/Slot_impl_fb ==
  frame_id : Inport  PortName=frame  Element=id
  frame_len : Inport  PortName=frame  Element=len
  frame_data : Inport  PortName=frame  Element=data
  frame_valid : Inport  PortName=frame  Element=valid
  drop : Inport  Port=2
  BC : BusCreator  Inputs=4  OutDataTypeStr=Bus: Bus_CanFrame8  NonVirtualBus=on
      settings: InheritFromInputs=off
  Held : UnitDelay  SampleTime=Ts.comm
  Hold : Switch  Criteria=u2 ~= 0  SaturateOnIntegerOverflow=off  InputSameDT=off
  Latency : Delay  DelayLength=P.electronics.can.can1_latency_samples  InitialCondition=P.ic.Bus_CanFrame8  SampleTime=Ts.comm
  NotDrop : Logic  Operator=NOT  Inputs=1  AllPortsSameDT=off  OutDataTypeStr=boolean
  Valid : Logic  AllPortsSameDT=off  OutDataTypeStr=boolean
  frame_rx : Outport
  wires:
  drop/1 -> NotDrop/1, Hold/2  "drop"
  frame_data/1 -> Hold/3  "data"
  NotDrop/1 -> Valid/2  "not_drop"
  Hold/1 -> BC/3, Held/1  "data_rx"
  frame_valid/1 -> Valid/1  "valid"
  Valid/1 -> BC/4  "valid_rx"
  Held/1 -> Hold/1  "data_held"
  frame_id/1 -> BC/1  "id"
  frame_len/1 -> BC/2  "len"
  BC/1 -> Latency/1  "frame_link"
  Latency/1 -> frame_rx/1  "frame_rx"

== system CAN1_Net_Sim/Slot_limits ==
  frame_id : Inport  PortName=frame  Element=id
  frame_len : Inport  PortName=frame  Element=len
  frame_data : Inport  PortName=frame  Element=data
  frame_valid : Inport  PortName=frame  Element=valid
  drop : Inport  Port=2
  BC : BusCreator  Inputs=4  OutDataTypeStr=Bus: Bus_CanFrame8  NonVirtualBus=on
      settings: InheritFromInputs=off
  Held : UnitDelay  SampleTime=Ts.hk
  Hold : Switch  Criteria=u2 ~= 0  SaturateOnIntegerOverflow=off  InputSameDT=off
  Latency : Delay  DelayLength=P.electronics.can.can1_latency_samples  InitialCondition=P.ic.Bus_CanFrame8  SampleTime=Ts.hk
  NotDrop : Logic  Operator=NOT  Inputs=1  AllPortsSameDT=off  OutDataTypeStr=boolean
  Valid : Logic  AllPortsSameDT=off  OutDataTypeStr=boolean
  frame_rx : Outport
  wires:
  drop/1 -> NotDrop/1, Hold/2  "drop"
  frame_data/1 -> Hold/3  "data"
  NotDrop/1 -> Valid/2  "not_drop"
  Hold/1 -> BC/3, Held/1  "data_rx"
  frame_valid/1 -> Valid/1  "valid"
  Valid/1 -> BC/4  "valid_rx"
  Held/1 -> Hold/1  "data_held"
  frame_id/1 -> BC/1  "id"
  frame_len/1 -> BC/2  "len"
  BC/1 -> Latency/1  "frame_link"
  Latency/1 -> frame_rx/1  "frame_rx"

== system CAN1_Net_Sim/Slot_power ==
  frame_id : Inport  PortName=frame  Element=id
  frame_len : Inport  PortName=frame  Element=len
  frame_data : Inport  PortName=frame  Element=data
  frame_valid : Inport  PortName=frame  Element=valid
  drop : Inport  Port=2
  BC : BusCreator  Inputs=4  OutDataTypeStr=Bus: Bus_CanFrame8  NonVirtualBus=on
      settings: InheritFromInputs=off
  Held : UnitDelay  SampleTime=Ts.hk
  Hold : Switch  Criteria=u2 ~= 0  SaturateOnIntegerOverflow=off  InputSameDT=off
  Latency : Delay  DelayLength=P.electronics.can.can1_latency_samples  InitialCondition=P.ic.Bus_CanFrame8  SampleTime=Ts.hk
  NotDrop : Logic  Operator=NOT  Inputs=1  AllPortsSameDT=off  OutDataTypeStr=boolean
  Valid : Logic  AllPortsSameDT=off  OutDataTypeStr=boolean
  frame_rx : Outport
  wires:
  drop/1 -> NotDrop/1, Hold/2  "drop"
  frame_data/1 -> Hold/3  "data"
  NotDrop/1 -> Valid/2  "not_drop"
  Hold/1 -> BC/3, Held/1  "data_rx"
  frame_valid/1 -> Valid/1  "valid"
  Valid/1 -> BC/4  "valid_rx"
  Held/1 -> Hold/1  "data_held"
  frame_id/1 -> BC/1  "id"
  frame_len/1 -> BC/2  "len"
  BC/1 -> Latency/1  "frame_link"
  Latency/1 -> frame_rx/1  "frame_rx"

== system CAN1_Net_Sim/Slot_soc ==
  frame_id : Inport  PortName=frame  Element=id
  frame_len : Inport  PortName=frame  Element=len
  frame_data : Inport  PortName=frame  Element=data
  frame_valid : Inport  PortName=frame  Element=valid
  drop : Inport  Port=2
  BC : BusCreator  Inputs=4  OutDataTypeStr=Bus: Bus_CanFrame8  NonVirtualBus=on
      settings: InheritFromInputs=off
  Held : UnitDelay  SampleTime=Ts.hk
  Hold : Switch  Criteria=u2 ~= 0  SaturateOnIntegerOverflow=off  InputSameDT=off
  Latency : Delay  DelayLength=P.electronics.can.can1_latency_samples  InitialCondition=P.ic.Bus_CanFrame8  SampleTime=Ts.hk
  NotDrop : Logic  Operator=NOT  Inputs=1  AllPortsSameDT=off  OutDataTypeStr=boolean
  Valid : Logic  AllPortsSameDT=off  OutDataTypeStr=boolean
  frame_rx : Outport
  wires:
  drop/1 -> NotDrop/1, Hold/2  "drop"
  frame_data/1 -> Hold/3  "data"
  NotDrop/1 -> Valid/2  "not_drop"
  Hold/1 -> BC/3, Held/1  "data_rx"
  frame_valid/1 -> Valid/1  "valid"
  Valid/1 -> BC/4  "valid_rx"
  Held/1 -> Hold/1  "data_held"
  frame_id/1 -> BC/1  "id"
  frame_len/1 -> BC/2  "len"
  BC/1 -> Latency/1  "frame_link"
  Latency/1 -> frame_rx/1  "frame_rx"

== system CAN1_Net_Sim/Slot_state ==
  frame_id : Inport  PortName=frame  Element=id
  frame_len : Inport  PortName=frame  Element=len
  frame_data : Inport  PortName=frame  Element=data
  frame_valid : Inport  PortName=frame  Element=valid
  drop : Inport  Port=2
  BC : BusCreator  Inputs=4  OutDataTypeStr=Bus: Bus_CanFrame8  NonVirtualBus=on
      settings: InheritFromInputs=off
  Held : UnitDelay  SampleTime=Ts.hk
  Hold : Switch  Criteria=u2 ~= 0  SaturateOnIntegerOverflow=off  InputSameDT=off
  Latency : Delay  DelayLength=P.electronics.can.can1_latency_samples  InitialCondition=P.ic.Bus_CanFrame8  SampleTime=Ts.hk
  NotDrop : Logic  Operator=NOT  Inputs=1  AllPortsSameDT=off  OutDataTypeStr=boolean
  Valid : Logic  AllPortsSameDT=off  OutDataTypeStr=boolean
  frame_rx : Outport
  wires:
  drop/1 -> NotDrop/1, Hold/2  "drop"
  frame_data/1 -> Hold/3  "data"
  NotDrop/1 -> Valid/2  "not_drop"
  Hold/1 -> BC/3, Held/1  "data_rx"
  frame_valid/1 -> Valid/1  "valid"
  Valid/1 -> BC/4  "valid_rx"
  Held/1 -> Hold/1  "data_held"
  frame_id/1 -> BC/1  "id"
  frame_len/1 -> BC/2  "len"
  BC/1 -> Latency/1  "frame_link"
  Latency/1 -> frame_rx/1  "frame_rx"

== system CAN1_Net_Sim/Slot_vit ==
  frame_id : Inport  PortName=frame  Element=id
  frame_len : Inport  PortName=frame  Element=len
  frame_data : Inport  PortName=frame  Element=data
  frame_valid : Inport  PortName=frame  Element=valid
  drop : Inport  Port=2
  BC : BusCreator  Inputs=4  OutDataTypeStr=Bus: Bus_CanFrame8  NonVirtualBus=on
      settings: InheritFromInputs=off
  Held : UnitDelay  SampleTime=Ts.hk
  Hold : Switch  Criteria=u2 ~= 0  SaturateOnIntegerOverflow=off  InputSameDT=off
  Latency : Delay  DelayLength=P.electronics.can.can1_latency_samples  InitialCondition=P.ic.Bus_CanFrame8  SampleTime=Ts.hk
  NotDrop : Logic  Operator=NOT  Inputs=1  AllPortsSameDT=off  OutDataTypeStr=boolean
  Valid : Logic  AllPortsSameDT=off  OutDataTypeStr=boolean
  frame_rx : Outport
  wires:
  drop/1 -> NotDrop/1, Hold/2  "drop"
  frame_data/1 -> Hold/3  "data"
  NotDrop/1 -> Valid/2  "not_drop"
  Hold/1 -> BC/3, Held/1  "data_rx"
  frame_valid/1 -> Valid/1  "valid"
  Valid/1 -> BC/4  "valid_rx"
  Held/1 -> Hold/1  "data_held"
  frame_id/1 -> BC/1  "id"
  frame_len/1 -> BC/2  "len"
  BC/1 -> Latency/1  "frame_link"
  Latency/1 -> frame_rx/1  "frame_rx"
